simulink model "Project1_Sim"  (R2022b)
settings: Solver=ode4  StartTime=0.0  StopTime=t_final  FixedStep=t_step  RelTol=1e-3
model workspace (MAT data in the model file):
  vel_0 = 0
values from neighbouring files (symbols this model uses):
  Ac = pi*0.125^2    (= 0.0490873852123)    [Project1.m]    (also in thrust.m = U(8))
  AOA = fsolve(fun,5)    [Fz_Fun.m]    (also in SLUF_Trim.m = sol(1); qs_Fun.m = U(3))
  beta = U(5)    [Force_Total.m]    (also in Fz_Fun.m = U(6); Project1.m = 0; qs_Fun.m = U(4))
  Ca = 5    [Project1.m]    (also in thrust.m = U(7))
  del_t = sol(2)    [SLUF_Trim.m]
  g = U(2)    [Fz_Fun.m]    (also in Project1.m = 9.81; ThreeDOF_Kinetics.m; qs_Fun.m; thrust.m = U(3))
  Isp = 50    [Project1.m]    (also in thrust.m = U(2))
  m = U(1)    [Fz_Fun.m]    (also in Project1.m = 2; ThreeDOF_Kinetics.m; qs_Fun.m)
  p = 0    [Project1.m]    (also in ThreeDOF_Kinetics.m = U(3))
  phi = 0    [Project1.m]    (also in ThreeDOF_Kinematics.m = U(5); ThreeDOF_Kinetics.m = U(10))
  pos_0 = [0;0;-alt_0-Re]    [Project1.m]
  psi = 0    [Project1.m]    (also in ThreeDOF_Kinematics.m = U(6))
  q = 0    [Project1.m]    (also in ThreeDOF_Kinetics.m = U(4))
  r = 0    [Project1.m]    (also in ThreeDOF_Kinetics.m = U(5))
  Re = 6.3781*10^6    (= 6378100)    [Project1.m]
  s = sind(angle)    [CoordinateTransform.m]    (also in Fz_Fun.m = U(5); Project1.m = 0.115824)
  theta = AOA    [Project1.m]    (also in SLUF_Trim.m; ThreeDOF_Kinematics.m = U(4); ThreeDOF_Kinetics.m = U(9))
  Vel_0 = [30;0;0]    [Project1.m]    (also in SLUF_Trim.m = [V*cosd(AOA);0;V*sind(AOA)])
undefined symbols (not defined in the file or in its folder): density, Force_Total, lift_drag_fun, magnitude, qs_Fun, speed_of_sound, ThreeDOF_Kinematics, ThreeDOF_Kinetics, thrust
settings Model: Creator=egger  LastModifiedBy=egger

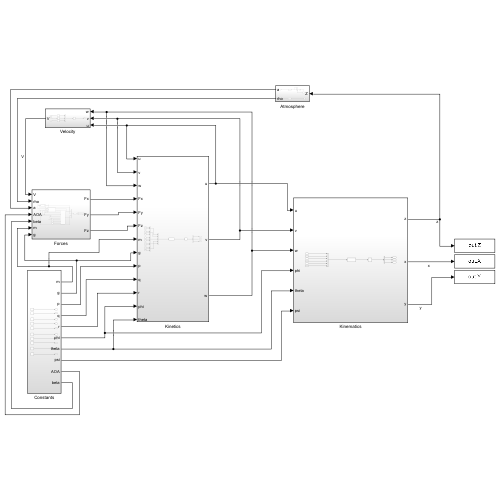
[thumbnail: Simulink's stored preview of the top-level diagram]
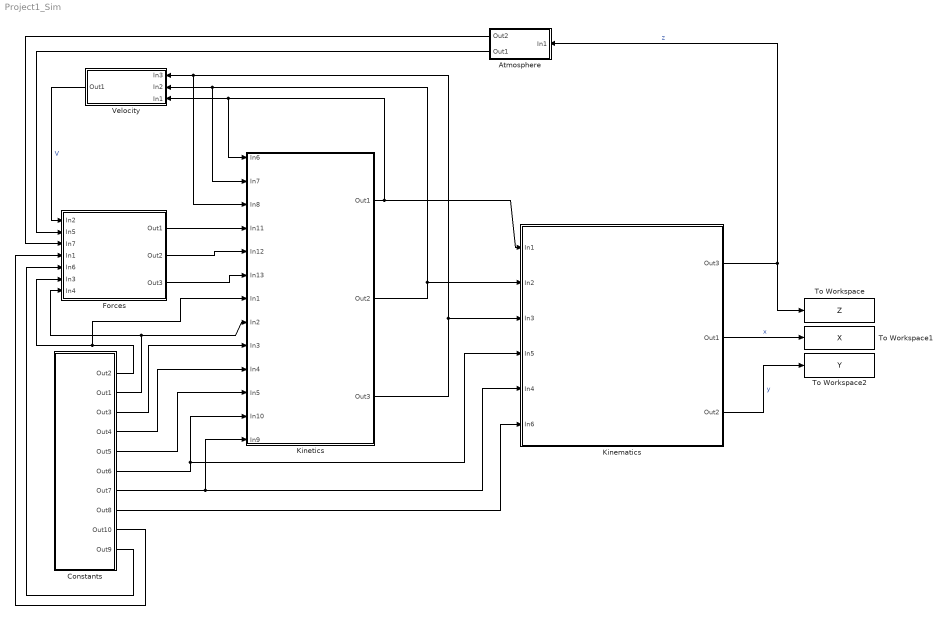
== system Project1_Sim ==
  Atmosphere : Subsystem
  Constants : Subsystem
  Forces : Subsystem
  Kinematics : Subsystem
  Kinetics : Subsystem
  To Workspace : ToWorkspace  VariableName=Z  SampleTime=-1
  To Workspace1 : ToWorkspace  VariableName=X  SampleTime=-1
  To Workspace2 : ToWorkspace  VariableName=Y  SampleTime=-1
  Velocity : Subsystem
  wires:
  Kinematics/2(Out1) -> To Workspace1/1  "x"
  Kinematics/1(Out3) -> To Workspace/1, Atmosphere/1(In1)  "z"
  Kinetics/1(Out1) -> Kinetics/1(In6), Velocity/3(In1), Kinematics/1(In1)
  Kinetics/2(Out2) -> Kinematics/2(In2), Kinetics/2(In7), Velocity/2(In2)
  Kinetics/3(Out3) -> Kinematics/3(In3), Kinetics/3(In8), Velocity/1(In3)
  Velocity/1(Out1) -> Forces/1(In2)  "V"
  Forces/1(Out1) -> Kinetics/4(In11)
  Forces/2(Out2) -> Kinetics/5(In12)
  Forces/3(Out3) -> Kinetics/6(In13)
  Atmosphere/2(Out1) -> Forces/2(In5)
  Atmosphere/1(Out2) -> Forces/3(In7)
  Constants/10(Out9) -> Forces/5(In6)
  Constants/9(Out10) -> Forces/4(In1)
  Constants/3(Out3) -> Kinetics/9(In3)
  Constants/4(Out4) -> Kinetics/10(In4)
  Constants/5(Out5) -> Kinetics/11(In5)
  Constants/7(Out7) -> Kinetics/13(In9), Kinematics/5(In4)
  Constants/6(Out6) -> Kinematics/4(In5), Kinetics/12(In10)
  Constants/1(Out2) -> Kinetics/7(In1), Forces/6(In3)
  Constants/2(Out1) -> Forces/7(In4), Kinetics/8(In2)
  Constants/8(Out8) -> Kinematics/6(In6)
  Kinematics/3(Out2) -> To Workspace2/1  "y"

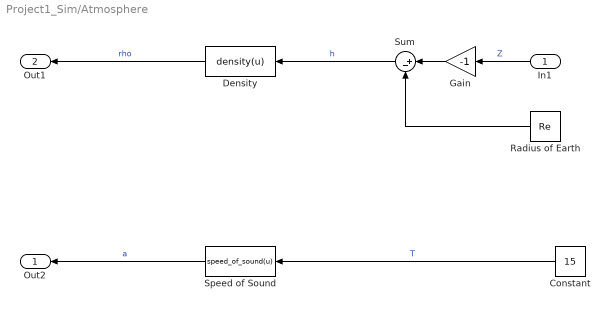
== system Project1_Sim/Atmosphere ==
  In1 : Inport
  Constant : Constant  Value=15
  Density : MATLABFcn  MATLABFcn=density(u)  OutputDimensions=1
  Gain : Gain  Gain=-1
  Radius of Earth : Constant  Value=Re
  Speed of Sound : MATLABFcn  MATLABFcn=speed_of_sound(u)  OutputDimensions=1
  Sum : Sum  Inputs=|+-
  Out2 : Outport
  Out1 : Outport  Port=2
  wires:
  In1/1 -> Gain/1  "Z"
  Radius of Earth/1 -> Sum/2
  Sum/1 -> Density/1  "h"
  Density/1 -> Out1/1  "rho"
  Constant/1 -> Speed of Sound/1  "T"
  Speed of Sound/1 -> Out2/1  "a"
  Gain/1 -> Sum/1

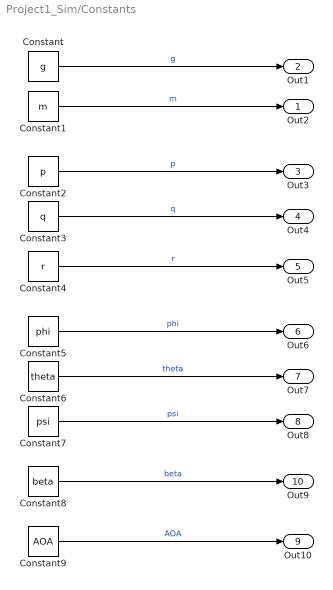
== system Project1_Sim/Constants ==
  Constant : Constant  Value=g
  Constant1 : Constant  Value=m
  Constant2 : Constant  Value=p
  Constant3 : Constant  Value=q
  Constant4 : Constant  Value=r
  Constant5 : Constant  Value=phi
  Constant6 : Constant  Value=theta
  Constant7 : Constant  Value=psi
  Constant8 : Constant  Value=beta
  Constant9 : Constant  Value=AOA
  Out2 : Outport
  Out1 : Outport  Port=2
  Out3 : Outport  Port=3
  Out4 : Outport  Port=4
  Out5 : Outport  Port=5
  Out6 : Outport  Port=6
  Out7 : Outport  Port=7
  Out8 : Outport  Port=8
  Out10 : Outport  Port=9
  Out9 : Outport  Port=10
  wires:
  Constant/1 -> Out1/1  "g"
  Constant1/1 -> Out2/1  "m"
  Constant2/1 -> Out3/1  "p"
  Constant3/1 -> Out4/1  "q"
  Constant4/1 -> Out5/1  "r"
  Constant5/1 -> Out6/1  "phi"
  Constant6/1 -> Out7/1  "theta"
  Constant7/1 -> Out8/1  "psi"
  Constant8/1 -> Out9/1  "beta"
  Constant9/1 -> Out10/1  "AOA"

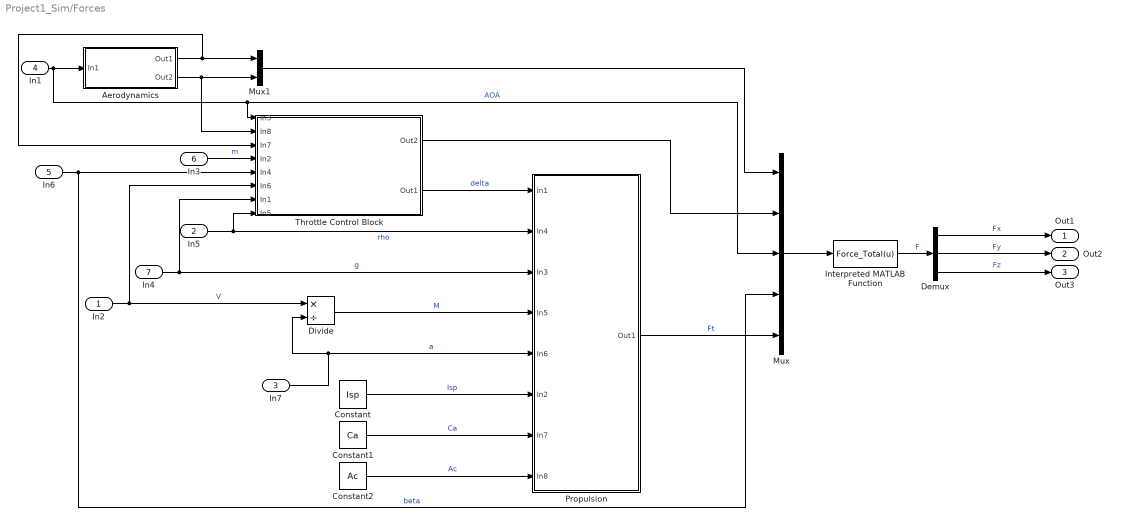
== system Project1_Sim/Forces ==
  In2 : Inport
  In5 : Inport  Port=2
  In7 : Inport  Port=3
  In1 : Inport  Port=4
  In6 : Inport  Port=5
  In3 : Inport  Port=6
  In4 : Inport  Port=7
  Aerodynamics : Subsystem
  Constant : Constant  Value=Isp
  Constant1 : Constant  Value=Ca
  Constant2 : Constant  Value=Ac
  Demux : Demux  Outputs=3
  Divide : Product  Inputs=*/
  Interpreted MATLAB Function : MATLABFcn  MATLABFcn=Force_Total(u)  OutputDimensions=3  OutputSignalType=real
  Mux : Mux  Inputs=5
  Mux1 : Mux  Inputs=2
  Propulsion : Subsystem
  Throttle Control Block : Subsystem
  Out1 : Outport
  Out2 : Outport  Port=2
  Out3 : Outport  Port=3
  wires:
  Mux/1 -> Interpreted MATLAB Function/1
  Interpreted MATLAB Function/1 -> Demux/1  "F"
  Demux/1 -> Out1/1  "Fx"
  Demux/2 -> Out2/1  "Fy"
  Demux/3 -> Out3/1  "Fz"
  Aerodynamics/1(Out1) -> Mux1/1, Throttle Control Block/3(In7)
  Aerodynamics/2(Out2) -> Mux1/2, Throttle Control Block/2(In8)
  Mux1/1 -> Mux/1
  Propulsion/1(Out1) -> Mux/5  "Ft"
  In1/1 -> Aerodynamics/1(In1), Mux/3, Throttle Control Block/1(In3)  "AOA"
  Constant/1 -> Propulsion/6(In2)  "Isp"
  In4/1 -> Throttle Control Block/7(In1), Propulsion/3(In3)  "g"
  Constant1/1 -> Propulsion/7(In7)  "Ca"
  Constant2/1 -> Propulsion/8(In8)  "Ac"
  Throttle Control Block/2(Out1) -> Propulsion/1(In1)  "delta"
  In2/1 -> Throttle Control Block/6(In6), Divide/1  "V"
  In5/1 -> Throttle Control Block/8(In5), Propulsion/2(In4)  "rho"
  In7/1 -> Propulsion/5(In6), Divide/2  "a"
  In3/1 -> Throttle Control Block/4(In2)  "m"
  In6/1 -> Mux/4, Throttle Control Block/5(In4)  "beta"
  Throttle Control Block/1(Out2) -> Mux/2
  Divide/1 -> Propulsion/4(In5)  "M"

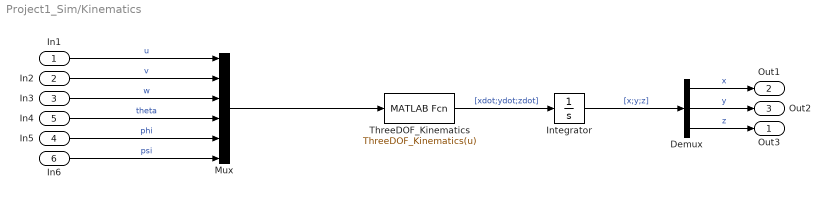
== system Project1_Sim/Kinematics ==
  In1 : Inport
  In2 : Inport  Port=2
  In3 : Inport  Port=3
  In5 : Inport  Port=4
  In4 : Inport  Port=5
  In6 : Inport  Port=6
  Demux : Demux  Outputs=3
  Integrator : Integrator  InitialCondition=pos_0
  Mux : Mux  Inputs=6
  ThreeDOF_Kinematics : MATLABFcn  MATLABFcn=ThreeDOF_Kinematics(u)  OutputDimensions=3
  Out3 : Outport
  Out1 : Outport  Port=2
  Out2 : Outport  Port=3
  wires:
  ThreeDOF_Kinematics/1 -> Integrator/1  "[xdot;ydot;zdot]"
  Integrator/1 -> Demux/1  "[x;y;z]"
  Mux/1 -> ThreeDOF_Kinematics/1
  In1/1 -> Mux/1  "u"
  In2/1 -> Mux/2  "v"
  In3/1 -> Mux/3  "w"
  In4/1 -> Mux/4  "theta"
  In5/1 -> Mux/5  "phi"
  In6/1 -> Mux/6  "psi"
  Demux/1 -> Out1/1  "x"
  Demux/2 -> Out2/1  "y"
  Demux/3 -> Out3/1  "z"

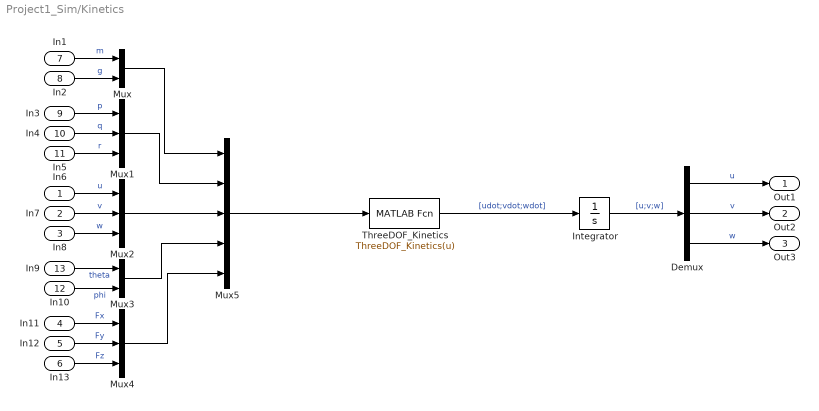
== system Project1_Sim/Kinetics ==
  In6 : Inport
  In7 : Inport  Port=2
  In8 : Inport  Port=3
  In11 : Inport  Port=4
  In12 : Inport  Port=5
  In13 : Inport  Port=6
  In1 : Inport  Port=7
  In2 : Inport  Port=8
  In3 : Inport  Port=9
  In4 : Inport  Port=10
  In5 : Inport  Port=11
  In10 : Inport  Port=12
  In9 : Inport  Port=13
  Demux : Demux  Outputs=3
  Integrator : Integrator  InitialCondition=Vel_0
  Mux : Mux  Inputs=2
  Mux1 : Mux  Inputs=3
  Mux2 : Mux  Inputs=3
  Mux3 : Mux  Inputs=2
  Mux4 : Mux  Inputs=3
  Mux5 : Mux  Inputs=5
  ThreeDOF_Kinetics : MATLABFcn  MATLABFcn=ThreeDOF_Kinetics(u)  OutputDimensions=3
  Out1 : Outport
  Out2 : Outport  Port=2
  Out3 : Outport  Port=3
  wires:
  Integrator/1 -> Demux/1  "[u;v;w]"
  Demux/1 -> Out1/1  "u"
  Demux/2 -> Out2/1  "v"
  Demux/3 -> Out3/1  "w"
  ThreeDOF_Kinetics/1 -> Integrator/1  "[udot;vdot;wdot]"
  In1/1 -> Mux/1  "m"
  In2/1 -> Mux/2  "g"
  In3/1 -> Mux1/1  "p"
  In4/1 -> Mux1/2  "q"
  In5/1 -> Mux1/3  "r"
  In6/1 -> Mux2/1  "u"
  In8/1 -> Mux2/3  "w"
  In7/1 -> Mux2/2  "v"
  In9/1 -> Mux3/1  "theta"
  In10/1 -> Mux3/2  "phi"
  In11/1 -> Mux4/1  "Fx"
  In13/1 -> Mux4/3  "Fz"
  In12/1 -> Mux4/2  "Fy"
  Mux/1 -> Mux5/1
  Mux1/1 -> Mux5/2
  Mux2/1 -> Mux5/3
  Mux3/1 -> Mux5/4
  Mux4/1 -> Mux5/5
  Mux5/1 -> ThreeDOF_Kinetics/1

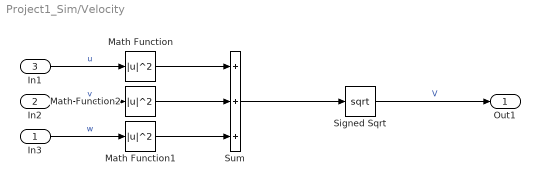
== system Project1_Sim/Velocity ==
  In3 : Inport
  In2 : Inport  Port=2
  In1 : Inport  Port=3
  Math Function : Math  Operator=magnitude^2
  Math Function1 : Math  Operator=magnitude^2
  Math Function2 : Math  Operator=magnitude^2
  Signed Sqrt : Sqrt  OutDataTypeStr=double
  Sum : Sum  Inputs=+++
  Out1 : Outport
  wires:
  In1/1 -> Math Function/1  "u"
  In2/1 -> Math Function2/1  "v"
  In3/1 -> Math Function1/1  "w"
  Math Function/1 -> Sum/1
  Math Function2/1 -> Sum/2
  Math Function1/1 -> Sum/3
  Sum/1 -> Signed Sqrt/1
  Signed Sqrt/1 -> Out1/1  "V"

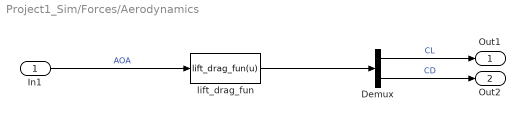
== system Project1_Sim/Forces/Aerodynamics ==
  In1 : Inport
  Demux : Demux  Outputs=2
  lift_drag_fun : MATLABFcn  MATLABFcn=lift_drag_fun(u)  OutputDimensions=2
  Out1 : Outport
  Out2 : Outport  Port=2
  wires:
  In1/1 -> lift_drag_fun/1  "AOA"
  lift_drag_fun/1 -> Demux/1
  Demux/1 -> Out1/1  "CL"
  Demux/2 -> Out2/1  "CD"

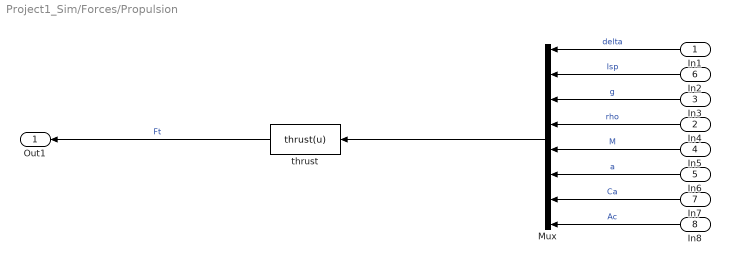
== system Project1_Sim/Forces/Propulsion ==
  In1 : Inport  OutDataTypeStr=fixdt('double', 'DataTypeOverride', 'Off')  LockScale=on
  In4 : Inport  Port=2
  In3 : Inport  Port=3
  In5 : Inport  Port=4
  In6 : Inport  Port=5
  In2 : Inport  Port=6
  In7 : Inport  Port=7
  In8 : Inport  Port=8
  Mux : Mux  Inputs=8
  thrust : MATLABFcn  MATLABFcn=thrust(u)  OutputDimensions=1
  Out1 : Outport
  wires:
  Mux/1 -> thrust/1
  thrust/1 -> Out1/1  "Ft"
  In1/1 -> Mux/1  "delta"
  In2/1 -> Mux/2  "Isp"
  In3/1 -> Mux/3  "g"
  In4/1 -> Mux/4  "rho"
  In5/1 -> Mux/5  "M"
  In6/1 -> Mux/6  "a"
  In7/1 -> Mux/7  "Ca"
  In8/1 -> Mux/8  "Ac"

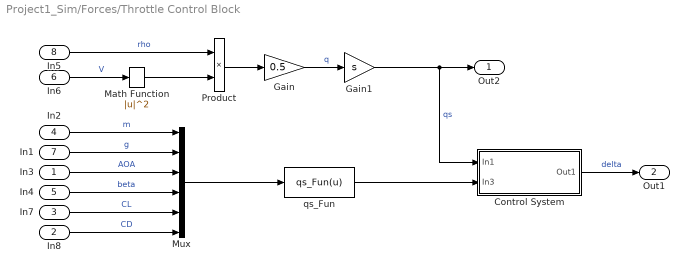
== system Project1_Sim/Forces/Throttle Control Block ==
  In3 : Inport
  In8 : Inport  Port=2
  In7 : Inport  Port=3
  In2 : Inport  Port=4
  In4 : Inport  Port=5
  In6 : Inport  Port=6
  In1 : Inport  Port=7
  In5 : Inport  Port=8
  Control System : Subsystem
  Gain : Gain  Gain=0.5  OutDataTypeStr=double
  Gain1 : Gain  Gain=s
  Math Function : Math  Operator=magnitude^2
  Mux : Mux  Inputs=6
  Product : Product  OutDataTypeStr=double  LockScale=on
  qs_Fun : MATLABFcn  MATLABFcn=qs_Fun(u)
  Out2 : Outport
  Out1 : Outport  Port=2  OutDataTypeStr=double  LockScale=on
  wires:
  In2/1 -> Mux/1  "m"
  In1/1 -> Mux/2  "g"
  In3/1 -> Mux/3  "AOA"
  In4/1 -> Mux/4  "beta"
  Mux/1 -> qs_Fun/1
  Gain/1 -> Gain1/1  "q"
  In6/1 -> Math Function/1  "V"
  Math Function/1 -> Product/2
  Product/1 -> Gain/1
  In5/1 -> Product/1  "rho"
  qs_Fun/1 -> Control System/2(In3)
  Control System/1(Out1) -> Out1/1  "delta"
  Gain1/1 -> Control System/1(In1), Out2/1  "qs"
  In8/1 -> Mux/6  "CD"
  In7/1 -> Mux/5  "CL"

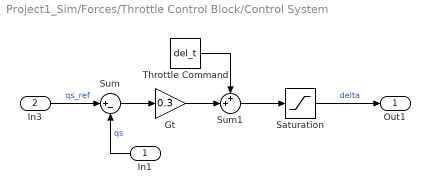
== system Project1_Sim/Forces/Throttle Control Block/Control System ==
  In1 : Inport
  In3 : Inport  Port=2
  Gt : Gain  Gain=0.3
  Saturation : Saturate  UpperLimit=1  LowerLimit=0  OutDataTypeStr=double
      settings: LockScale=on
  Sum : Sum  Inputs=|+-
  Sum1 : Sum  Inputs=++|
  Throttle Command : Constant  Value=del_t
  Out1 : Outport
  wires:
  Saturation/1 -> Out1/1  "delta"
  In3/1 -> Sum/1  "qs_ref"
  Sum/1 -> Gt/1
  Gt/1 -> Sum1/2
  Throttle Command/1 -> Sum1/1
  Sum1/1 -> Saturation/1
  In1/1 -> Sum/2  "qs"
